simulink model "CruiseControl_Simul2"  (R2022b)
settings: Solver=FixedStepAuto  StartTime=0.0  StopTime=10  FixedStep=0.0001  RelTol=1e-3
values from neighbouring files (symbols this model uses):
  Af = 4    [CruiseControl_Initialize.m]
  C_long = 6*10^4    (= 60000)    [CruiseControl_Initialize.m]
  Cd = 0.3    [CruiseControl_Initialize.m]
  g = 9.81    [CruiseControl_Initialize.m]
  I_wheel = 0.8    [CruiseControl_Initialize.m]
  K_I = 0.01    [CruiseControl_Initialize.m]
  K_P = 0.1    [CruiseControl_Initialize.m]
  m = 1500    [CruiseControl_Initialize.m]
  r_eff = rw * sin(phi)/phi    [CruiseControl_Initialize.m]
  R_roll = 0.015    [CruiseControl_Initialize.m]
  rho = 1.225    [CruiseControl_Initialize.m]
  V_desire = 100    [CruiseControl_Initialize.m]
  x_0 = 0    [CruiseControl_Initialize.m]
  xdot_0 = 60    [CruiseControl_Initialize.m]
settings Model: Creator=lego0  LastModifiedBy=lego0

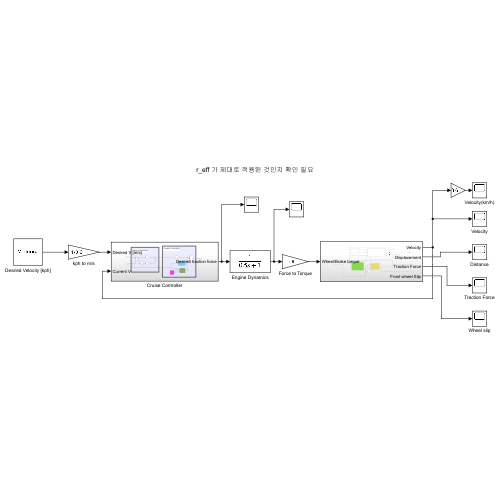
[thumbnail: Simulink's stored preview of the top-level diagram]
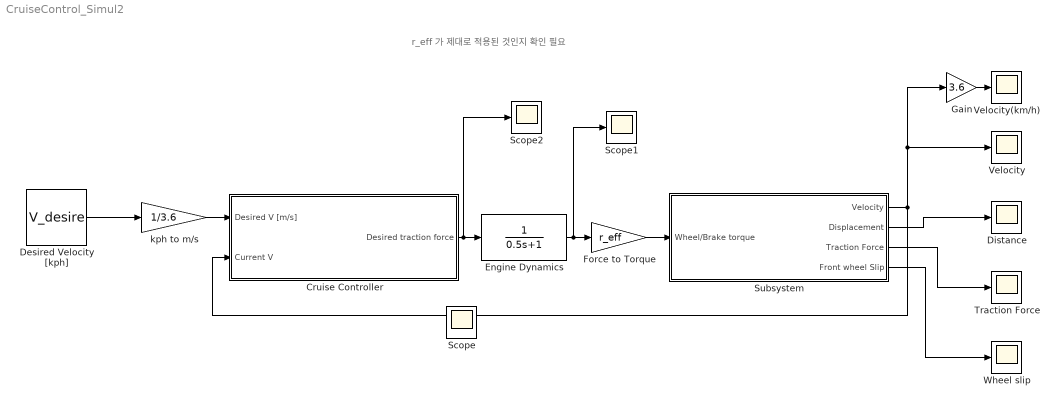
== system CruiseControl_Simul2 ==
  note: r_eff 가 제대로 적용된 것인지 확인 필요
  Cruise Controller : Subsystem
  Desired Velocity [kph] : Constant  Value=V_desire
  Distance : Scope
  Engine Dynamics : TransferFcn  Denominator=[0.5 1]
  Force to Torque : Gain  Gain=r_eff
  Gain : Gain  Gain=3.6
  Scope1 : Scope
  Scope2 : Scope
  Subsystem : Subsystem
  Traction Force : Scope
  Velocity : Scope
  Velocity(km/h) : Scope
  Wheel slip : Scope
  kph to m/s : Gain  Gain=1/3.6
  Scope : Scope
  wires:
  Gain/1 -> Velocity(km/h)/1
  Cruise Controller/1(Desired traction force) -> Scope2/1, Engine Dynamics/1
  Desired Velocity [kph]/1 -> kph to m/s/1
  kph to m/s/1 -> Cruise Controller/1(Desired V [m/s])
  Subsystem/1(Velocity) -> Cruise Controller/2(Current V), Gain/1, Velocity/1
  Subsystem/2(Displacement) -> Distance/1
  Subsystem/3(Traction Force) -> Traction Force/1
  Subsystem/4(Front wheel Slip) -> Wheel slip/1
  Engine Dynamics/1 -> Scope1/1, Force to Torque/1
  Force to Torque/1 -> Subsystem/1(Wheel/Brake torque)

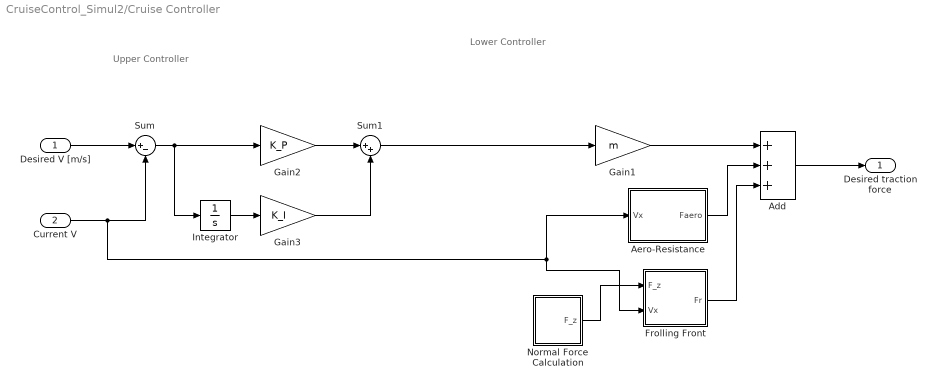
== system CruiseControl_Simul2/Cruise Controller ==
  note: Upper Controller
  note: Lower Controller
  Desired V [m/s] : Inport
  Current V : Inport  Port=2
  Add : Sum  Inputs=+++
  Aero-Resistance : Subsystem
  Frolling Front : Subsystem
  Gain1 : Gain  Gain=m
  Gain2 : Gain  Gain=K_P
  Gain3 : Gain  Gain=K_I
  Integrator : Integrator
  Normal Force Calculation : Subsystem
  Sum : Sum  Inputs=|+-
  Sum1 : Sum  Inputs=|++
  Desired traction force : Outport
  wires:
  Gain2/1 -> Sum1/1
  Current V/1 -> Frolling Front/2(Vx), Aero-Resistance/1(Vx), Sum/2
  Gain3/1 -> Sum1/2
  Sum/1 -> Integrator/1, Gain2/1
  Integrator/1 -> Gain3/1
  Desired V [m/s]/1 -> Sum/1
  Sum1/1 -> Gain1/1
  Gain1/1 -> Add/1
  Add/1 -> Desired traction force/1
  Normal Force Calculation/1(F_z) -> Frolling Front/1(F_z)
  Aero-Resistance/1(Faero) -> Add/2
  Frolling Front/1(Fr) -> Add/3

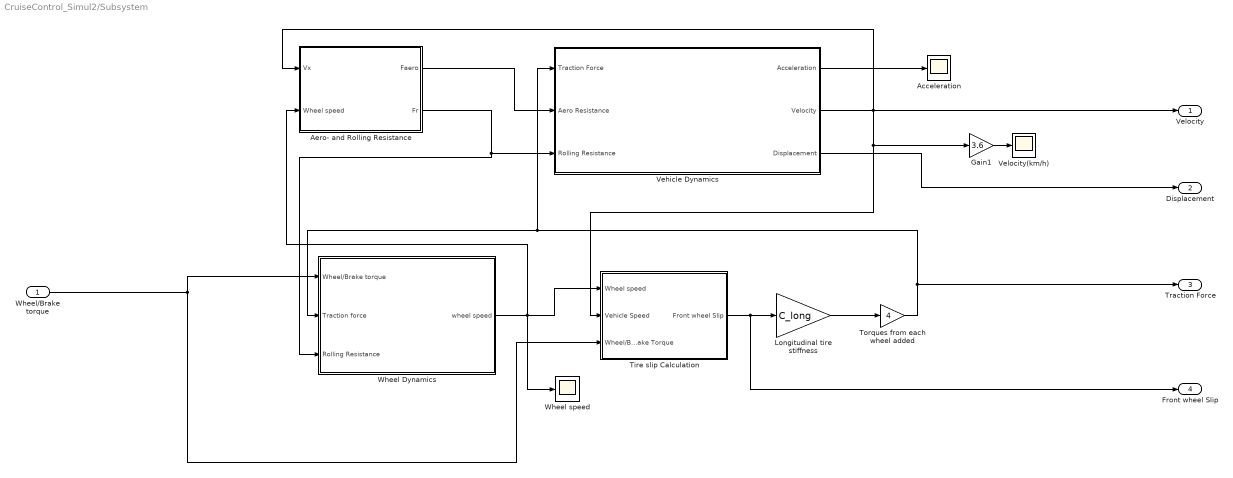
== system CruiseControl_Simul2/Subsystem ==
  Wheel/Brake torque : Inport
  Acceleration : Scope
  Aero- and Rolling Resistance : Subsystem
  Gain1 : Gain  Gain=3.6
  Longitudinal tire stiffness : Gain  Gain=C_long
  Tire slip Calculation : Subsystem
  Torques from each wheel added : Gain  Gain=4
  Vehicle Dynamics : Subsystem
  Velocity(km/h) : Scope
  Wheel Dynamics : Subsystem
  Wheel speed : Scope
  Velocity : Outport
  Displacement : Outport  Port=2
  Traction Force : Outport  Port=3
  Front wheel Slip : Outport  Port=4
  wires:
  Wheel Dynamics/1(wheel speed) -> Wheel speed/1, Aero- and Rolling Resistance/2(Wheel speed), Tire slip Calculation/1(Wheel speed)
  Torques from each wheel added/1 -> Traction Force/1, Vehicle Dynamics/1(Traction Force), Wheel Dynamics/2(Traction force)
  Longitudinal tire stiffness/1 -> Torques from each wheel added/1
  Aero- and Rolling Resistance/2(Fr) -> Wheel Dynamics/3(Rolling Resistance), Vehicle Dynamics/3(Rolling Resistance)
  Vehicle Dynamics/2(Velocity) -> Velocity/1, Tire slip Calculation/2(Vehicle Speed), Gain1/1, Aero- and Rolling Resistance/1(Vx)
  Tire slip Calculation/1(Front wheel Slip) -> Front wheel Slip/1, Longitudinal tire stiffness/1
  Aero- and Rolling Resistance/1(Faero) -> Vehicle Dynamics/2(Aero Resistance)
  Vehicle Dynamics/1(Acceleration) -> Acceleration/1
  Gain1/1 -> Velocity(km/h)/1
  Vehicle Dynamics/3(Displacement) -> Displacement/1
  Wheel/Brake torque/1 -> Wheel Dynamics/1(Wheel/Brake torque), Tire slip Calculation/3(Wheel/Brake Torque)

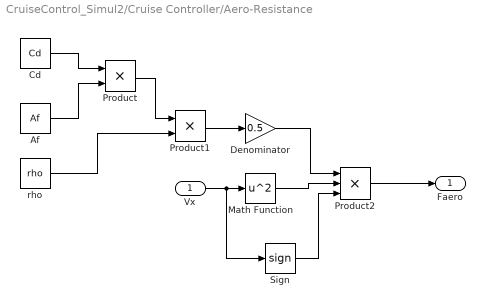
== system CruiseControl_Simul2/Cruise Controller/Aero-Resistance ==
  Vx : Inport
  Af : Constant  Value=Af
  Cd : Constant  Value=Cd
  Denominator : Gain  Gain=0.5
  Math Function : Math  Operator=square  SignedPower=on
  Product : Product
  Product1 : Product
  Product2 : Product  Inputs=3
  Sign : Signum
  rho : Constant  Value=rho
  Faero : Outport  VectorParamsAs1DForOutWhenUnconnected=off
  wires:
  Af/1 -> Product/2
  Product1/1 -> Denominator/1
  Denominator/1 -> Product2/1
  Vx/1 -> Sign/1, Math Function/1
  rho/1 -> Product1/2
  Cd/1 -> Product/1
  Math Function/1 -> Product2/2
  Product/1 -> Product1/1
  Sign/1 -> Product2/3
  Product2/1 -> Faero/1

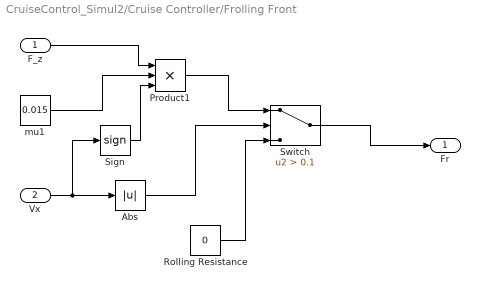
== system CruiseControl_Simul2/Cruise Controller/Frolling Front ==
  F_z : Inport
  Vx : Inport  Port=2
  Abs : Abs  SaturateOnIntegerOverflow=off
  Product1 : Product  Inputs=3
  Rolling Resistance : Constant  Value=0
  Sign : Signum
  Switch : Switch  Criteria=u2 > Threshold  Threshold=0.1  SaturateOnIntegerOverflow=off  InputSameDT=off
  mu1 : Constant  Value=0.015
  Fr : Outport  VectorParamsAs1DForOutWhenUnconnected=off
  wires:
  F_z/1 -> Product1/1
  Product1/1 -> Switch/1
  Rolling Resistance/1 -> Switch/3
  mu1/1 -> Product1/2
  Vx/1 -> Sign/1, Abs/1
  Abs/1 -> Switch/2
  Sign/1 -> Product1/3
  Switch/1 -> Fr/1

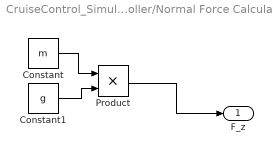
== system CruiseControl_Simul2/Cruise Controller/Normal Force Calculation ==
  Constant : Constant  Value=m
  Constant1 : Constant  Value=g
  Product : Product
  F_z : Outport
  wires:
  Product/1 -> F_z/1
  Constant1/1 -> Product/2
  Constant/1 -> Product/1

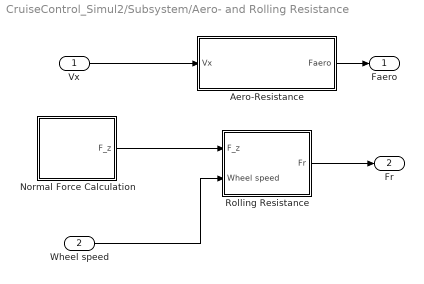
== system CruiseControl_Simul2/Subsystem/Aero- and Rolling Resistance ==
  Vx : Inport
  Wheel speed : Inport  Port=2
  Aero-Resistance : Subsystem
  Normal Force Calculation : Subsystem
  Rolling Resistance : Subsystem
  Faero : Outport
  Fr : Outport  Port=2
  wires:
  Rolling Resistance/1(Fr) -> Fr/1
  Normal Force Calculation/1(F_z) -> Rolling Resistance/1(F_z)
  Vx/1 -> Aero-Resistance/1(Vx)
  Wheel speed/1 -> Rolling Resistance/2(Wheel speed)
  Aero-Resistance/1(Faero) -> Faero/1

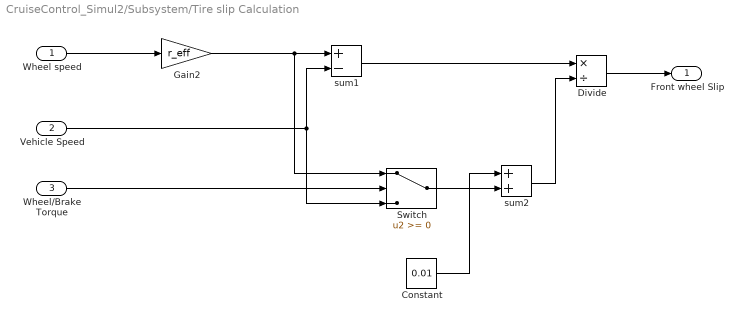
== system CruiseControl_Simul2/Subsystem/Tire slip Calculation ==
  Wheel speed : Inport
  Vehicle Speed : Inport  Port=2
  Wheel/Brake Torque : Inport  Port=3
  Constant : Constant  Value=0.01
  Divide : Product  Inputs=*/
  Gain2 : Gain  Gain=r_eff
  Switch : Switch  SaturateOnIntegerOverflow=off  InputSameDT=off
  sum1 : Sum  Inputs=+-
  sum2 : Sum
  Front wheel Slip : Outport  VectorParamsAs1DForOutWhenUnconnected=off
  wires:
  Vehicle Speed/1 -> sum1/2, Switch/3
  Gain2/1 -> Switch/1, sum1/1
  Wheel speed/1 -> Gain2/1
  sum1/1 -> Divide/1
  Divide/1 -> Front wheel Slip/1
  Switch/1 -> sum2/2
  sum2/1 -> Divide/2
  Constant/1 -> sum2/1
  Wheel/Brake Torque/1 -> Switch/2

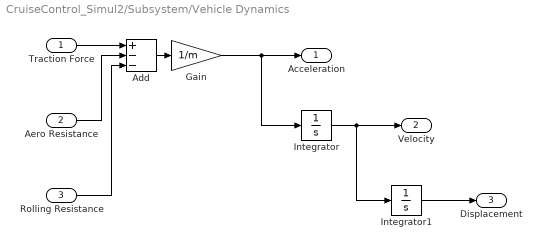
== system CruiseControl_Simul2/Subsystem/Vehicle Dynamics ==
  Traction Force : Inport
  Aero Resistance : Inport  Port=2
  Rolling Resistance : Inport  Port=3
  Add : Sum  Inputs=+--
  Gain : Gain  Gain=1/m
  Integrator : Integrator  InitialCondition=xdot_0/3.6
  Integrator1 : Integrator  InitialCondition=x_0
  Acceleration : Outport
  Velocity : Outport  Port=2
  Displacement : Outport  Port=3
  wires:
  Integrator1/1 -> Displacement/1
  Gain/1 -> Integrator/1, Acceleration/1
  Integrator/1 -> Integrator1/1, Velocity/1
  Add/1 -> Gain/1
  Traction Force/1 -> Add/1
  Aero Resistance/1 -> Add/2
  Rolling Resistance/1 -> Add/3

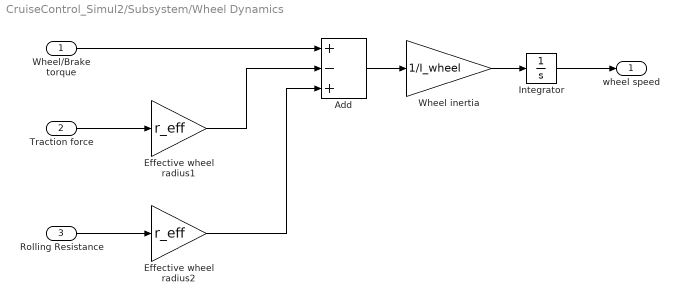
== system CruiseControl_Simul2/Subsystem/Wheel Dynamics ==
  Wheel/Brake torque : Inport
  Traction force : Inport  Port=2
  Rolling Resistance : Inport  Port=3
  Add : Sum  Inputs=+-+
  Effective wheel radius1 : Gain  Gain=r_eff
  Effective wheel radius2 : Gain  Gain=r_eff
  Integrator : Integrator
  Wheel inertia : Gain  Gain=1/I_wheel
  wheel speed : Outport
  wires:
  Wheel inertia/1 -> Integrator/1
  Integrator/1 -> wheel speed/1
  Add/1 -> Wheel inertia/1
  Wheel/Brake torque/1 -> Add/1
  Traction force/1 -> Effective wheel radius1/1
  Rolling Resistance/1 -> Effective wheel radius2/1
  Effective wheel radius1/1 -> Add/2
  Effective wheel radius2/1 -> Add/3

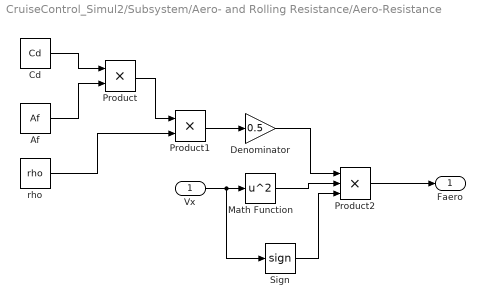
== system CruiseControl_Simul2/Subsystem/Aero- and Rolling Resistance/Aero-Resistance ==
  Vx : Inport
  Af : Constant  Value=Af
  Cd : Constant  Value=Cd
  Denominator : Gain  Gain=0.5
  Math Function : Math  Operator=square  SignedPower=on
  Product : Product
  Product1 : Product
  Product2 : Product  Inputs=3
  Sign : Signum
  rho : Constant  Value=rho
  Faero : Outport  VectorParamsAs1DForOutWhenUnconnected=off
  wires:
  Af/1 -> Product/2
  Product1/1 -> Denominator/1
  Denominator/1 -> Product2/1
  Vx/1 -> Sign/1, Math Function/1
  rho/1 -> Product1/2
  Cd/1 -> Product/1
  Math Function/1 -> Product2/2
  Product/1 -> Product1/1
  Sign/1 -> Product2/3
  Product2/1 -> Faero/1

== system CruiseControl_Simul2/Subsystem/Aero- and Rolling Resistance/Normal Force Calculation ==
  Constant : Constant  Value=m
  Constant1 : Constant  Value=g
  Product : Product
  F_z : Outport
  wires:
  Product/1 -> F_z/1
  Constant1/1 -> Product/2
  Constant/1 -> Product/1

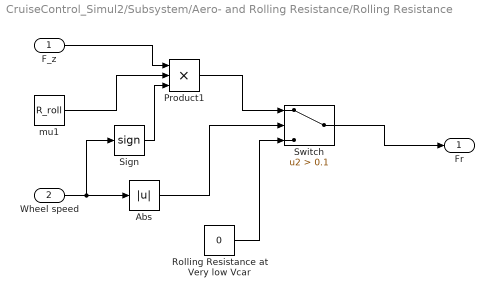
== system CruiseControl_Simul2/Subsystem/Aero- and Rolling Resistance/Rolling Resistance ==
  F_z : Inport
  Wheel speed : Inport  Port=2
  Abs : Abs  SaturateOnIntegerOverflow=off
  Product1 : Product  Inputs=3
  Rolling Resistance at Very low Vcar : Constant  Value=0
  Sign : Signum
  Switch : Switch  Criteria=u2 > Threshold  Threshold=0.1  SaturateOnIntegerOverflow=off  InputSameDT=off
  mu1 : Constant  Value=R_roll
  Fr : Outport  VectorParamsAs1DForOutWhenUnconnected=off
  wires:
  F_z/1 -> Product1/1
  Product1/1 -> Switch/1
  Rolling Resistance at Very low Vcar/1 -> Switch/3
  mu1/1 -> Product1/2
  Wheel speed/1 -> Sign/1, Abs/1
  Abs/1 -> Switch/2
  Sign/1 -> Product1/3
  Switch/1 -> Fr/1
